simulink model "Full_Car_Model"  (R2023b)
settings: Solver=FixedStepAuto  StartTime=0.0  StopTime=t_end_sim  FixedStep=Ts_sim  RelTol=1e-3
values from neighbouring files (symbols this model uses):
  a_b_ref_sat = [ zeros(1,10) ... (first row only)    [A1_Init.m]    (also in C1_MonteCarloAnalysis.m)
  adaptive = 3    [A1_Init.m]    (also in C1_MonteCarloAnalysis.m = 1)
  data = A2_Full_car_model_parameters_4onBoard()    [A1_Init.m]    (also in C1_MonteCarloAnalysis.m)
  Ft_demand_F = [zeros(1,601) 200*ones(1,2400)]./data.R_F    [A1_Init.m]    (also in C1_MonteCarloAnalysis.m)
  Ft_demand_R = [zeros(1,(601-length(l_discr)))              200*ones(1,(2400+length(l_discr)))]./data.R_R    [A1_Init.m]    (also in C1_MonteCarloAnalysis.m)
  handmade_front = strcat(currentPath,'\Road_profiles\height_crg_files\','handmade_step_3cm_singlefunctions.crg')    [A1_Init.m]    (also in C1_MonteCarloAnalysis.m)
  handmade_mu_front = strcat(currentPath,'\Road_profiles\friction_crg_files\','handmade_fric_step_01_singlefunctions.crg')    [A1_Init.m]    (also in C1_MonteCarloAnalysis.m)
  handmade_mu_rear = handmade_mu_front    [A1_Init.m]    (also in C1_MonteCarloAnalysis.m)
  handmade_rear = handmade_front    [A1_Init.m]    (also in C1_MonteCarloAnalysis.m)
  LowLim_Q1 = -10    [A1_Init.m]    (also in C1_MonteCarloAnalysis.m)
  M = N    (= 10)    [A1_Init.m]    (also in C1_MonteCarloAnalysis.m)
  mu_distance = test_distance    [A1_Init.m]    (also in C1_MonteCarloAnalysis.m)
  mu_road = [ones(1,1001), 0.1*ones(1,2000)]    [A1_Init.m]    (also in C1_MonteCarloAnalysis.m)
  N = 10    [A1_Init.m]    (also in C1_MonteCarloAnalysis.m)
  N_iter = 3    [A1_Init.m]    (also in C1_MonteCarloAnalysis.m)
  omega_ini_F_L = x_u_dot_ini_F_L/data.R_F    [A1_Init.m]    (also in C1_MonteCarloAnalysis.m)
  omega_ini_F_R = x_u_dot_ini_R_R/data.R_F    [A1_Init.m]    (also in C1_MonteCarloAnalysis.m)
  omega_ini_R_L = x_u_dot_ini_R_L/data.R_R +2.483*1e-6    [A1_Init.m]    (also in C1_MonteCarloAnalysis.m)
  omega_ini_R_R = x_u_dot_ini_R_R/data.R_R+2.483*1e-6    [A1_Init.m]    (also in C1_MonteCarloAnalysis.m)
  passive = 2    [A1_Init.m]    (also in C1_MonteCarloAnalysis.m)
  Pitch = 0    [A1_Init.m]    (also in C1_MonteCarloAnalysis.m)
  Pitch_dot = 0    [A1_Init.m]    (also in C1_MonteCarloAnalysis.m)
  preview = 2    [A1_Init.m]    (also in C1_MonteCarloAnalysis.m)
  Q1 = 1e6    (= 1000000)    [A1_Init.m]    (also in C1_MonteCarloAnalysis.m)
  Q1_sat = 0    [A1_Init.m]    (also in C1_MonteCarloAnalysis.m)
  Q2 = 1e5    (= 100000)    [A1_Init.m]    (also in C1_MonteCarloAnalysis.m)
  QN1 = 0    [A1_Init.m]    (also in C1_MonteCarloAnalysis.m)
  QN2 = 0    [A1_Init.m]    (also in C1_MonteCarloAnalysis.m)
  R1 = 1e10    (= 10000000000)    [A1_Init.m]    (also in C1_MonteCarloAnalysis.m)
  r1_h0 = 0.99    [A1_Init.m]    (also in C1_MonteCarloAnalysis.m)
  r1_k = 1000    [A1_Init.m]    (also in C1_MonteCarloAnalysis.m)
  r1_max = 11    [A1_Init.m]    (also in C1_MonteCarloAnalysis.m)
  r1_min = -10    [A1_Init.m]    (also in C1_MonteCarloAnalysis.m)
  r2 = 2    [A1_Init.m]    (also in C1_MonteCarloAnalysis.m)
  R2 = 1e2    (= 100)    [A1_Init.m]    (also in C1_MonteCarloAnalysis.m)
  R2_rl = 2    [A1_Init.m]    (also in C1_MonteCarloAnalysis.m)
  road_profile = [zeros(1,801),ones(1,2200)*10*Step_selector]    [A1_Init.m]    (also in C1_MonteCarloAnalysis.m)
  T_distance = test_distance    [A1_Init.m]    (also in C1_MonteCarloAnalysis.m)
  T_hs_ini_F_L = 0    [A1_Init.m]    (also in C1_MonteCarloAnalysis.m)
  T_hs_ini_F_R = 0    [A1_Init.m]    (also in C1_MonteCarloAnalysis.m)
  T_hs_ini_R_L = 0    [A1_Init.m]    (also in C1_MonteCarloAnalysis.m)
  T_hs_ini_R_R = 0    [A1_Init.m]    (also in C1_MonteCarloAnalysis.m)
  test_distance = 0:0.01:30    [A1_Init.m]    (also in C1_MonteCarloAnalysis.m)
  theta_s_ini_F_L = 0    [A1_Init.m]    (also in C1_MonteCarloAnalysis.m)
  theta_s_ini_F_R = 0    [A1_Init.m]    (also in C1_MonteCarloAnalysis.m)
  theta_s_ini_R_L = 0    [A1_Init.m]    (also in C1_MonteCarloAnalysis.m)
  theta_s_ini_R_R = 0    [A1_Init.m]    (also in C1_MonteCarloAnalysis.m)
  theta_w_ini_F_L = -1.056*1e-2    (= -0.01056)    [A1_Init.m]    (also in C1_MonteCarloAnalysis.m)
  theta_w_ini_R_L = -1.056*1e-2    (= -0.01056)    [A1_Init.m]    (also in C1_MonteCarloAnalysis.m)
  Ts = 1e-3*[0 5 10 15 20 25 30 40 60 80 100]    [A1_Init.m]    (also in C1_MonteCarloAnalysis.m)
  w1_h0 = 0.0008    [A1_Init.m]    (also in C1_MonteCarloAnalysis.m)
  w1_k = 5000    [A1_Init.m]    (also in C1_MonteCarloAnalysis.m)
  w1_max = 9    [A1_Init.m]    (also in C1_MonteCarloAnalysis.m)
  w1_min = -10    [A1_Init.m]    (also in C1_MonteCarloAnalysis.m)
  w1_sat = 0.085    [A1_Init.m]    (also in C1_MonteCarloAnalysis.m)
  w2_h0 = 2    [A1_Init.m]    (also in C1_MonteCarloAnalysis.m)
  w2_inc = 0.05    [A1_Init.m]    (also in C1_MonteCarloAnalysis.m)
  w2_k = 10    [A1_Init.m]    (also in C1_MonteCarloAnalysis.m)
  w2_max = 5.3    [A1_Init.m]    (also in C1_MonteCarloAnalysis.m)
  w2_min = -10    [A1_Init.m]    (also in C1_MonteCarloAnalysis.m)
  Wmat_NMPC_init = [W(1,:) W(2,:) W(3,:) W(4,:)]    [A1_Init.m]    (also in C1_MonteCarloAnalysis.m)
  WNmat_NMPC_init = [WN(1,:) WN(2,:)]    [A1_Init.m]    (also in C1_MonteCarloAnalysis.m)
  X_0 = [z_b_dot_ini z_b_ini z_u_dot_ini_F_L z_u_ini_F_L x_b_dot_ini x_b_ini x_u_dot_ini_F_L x_u_ini_F_L          omega_ini_F_L theta_w_ini_F_L omega_ini_F_L theta_s_ini_F_L torque_ini_F_L]    [A1_Init.m]    (also in C1_MonteCarloAnalysis.m)
  x_b_dot_ini = speed_ini/3.6    (= 11.1111111111)    [A1_Init.m]    (also in C1_MonteCarloAnalysis.m)
  x_b_ini = data.b+pos_ini    [A1_Init.m]    (also in C1_MonteCarloAnalysis.m)
  x_u_dot_ini_F_L = speed_ini/3.6 - 1.125*1e-4    (= 11.1109986111)    [A1_Init.m]    (also in C1_MonteCarloAnalysis.m)
  x_u_dot_ini_F_R = speed_ini/3.6 - 1.125*1e-4    (= 11.1109986111)    [A1_Init.m]    (also in C1_MonteCarloAnalysis.m)
  x_u_dot_ini_R_L = speed_ini/3.6 - 1.125*1e-4    (= 11.1109986111)    [A1_Init.m]    (also in C1_MonteCarloAnalysis.m)
  x_u_dot_ini_R_R = speed_ini/3.6 - 1.125*1e-4    (= 11.1109986111)    [A1_Init.m]    (also in C1_MonteCarloAnalysis.m)
  x_u_ini_F_L = data.a+data.b+pos_ini    [A1_Init.m]    (also in C1_MonteCarloAnalysis.m)
  x_u_ini_F_R = data.a+data.b+pos_ini    [A1_Init.m]    (also in C1_MonteCarloAnalysis.m)
  x_u_ini_R_L = pos_ini    (= 0)    [A1_Init.m]    (also in C1_MonteCarloAnalysis.m)
  x_u_ini_R_R = pos_ini    (= 0)    [A1_Init.m]    (also in C1_MonteCarloAnalysis.m)
  z_b_dot_ini = 0    [A1_Init.m]    (also in C1_MonteCarloAnalysis.m)
  z_b_ini = 0    [A1_Init.m]    (also in C1_MonteCarloAnalysis.m)
  z_u_dot_ini_F_L = 0    [A1_Init.m]    (also in C1_MonteCarloAnalysis.m)
  z_u_dot_ini_F_R = 0    [A1_Init.m]    (also in C1_MonteCarloAnalysis.m)
  z_u_dot_ini_R_L = 0    [A1_Init.m]    (also in C1_MonteCarloAnalysis.m)
  z_u_dot_ini_R_R = 0    [A1_Init.m]    (also in C1_MonteCarloAnalysis.m)
  z_u_ini_F_L = 0    [A1_Init.m]    (also in C1_MonteCarloAnalysis.m)
  z_u_ini_F_R = 0    [A1_Init.m]    (also in C1_MonteCarloAnalysis.m)
  z_u_ini_R_L = 0    [A1_Init.m]    (also in C1_MonteCarloAnalysis.m)
  z_u_ini_R_R = 0    [A1_Init.m]    (also in C1_MonteCarloAnalysis.m)
undefined symbols (not defined in the file or in its folder): Delay_step, road_with_noise
libraries: mfswift_library x8, rllib x4, simulink x4
(part 6 of 7)

== matlab function Full_Car_Model/CONTROLLER REAR RIGHT/ROAD PREVIEW/ROAD PREVIEW ==
  data: w input; OnlineData output; beta_y input; Tm_req input; Tm_req_R2 input; Tm_req_F_L input; Tm_req_F_R input; N parameter; M parameter; mu_act input; sigma_ref input
function OnlineData=OnlineDataArray(w, beta_y, Tm_req, Tm_req_R2, Tm_req_F_L, Tm_req_F_R, N, M, mu_act, sigma_ref)

OnlineData = repmat([0; 0; Tm_req; Tm_req_R2; Tm_req_F_L; Tm_req_F_R; 0; 0],N+1,1);

for i = 1:M+1       % M = Time preview steps
    OnlineData(8*i-7) = w(i);
    OnlineData(8*i-6) = beta_y(i);
    OnlineData(8*i-1) = mu_act(i);
    OnlineData(8*i) = sigma_ref(i);
end

for i = M+2:N+1     % N = Time horizon steps
    OnlineData(8*i-7) = w(end);
    OnlineData(8*i-6) = beta_y(end);
    OnlineData(8*i-1) = mu_act(end);
    OnlineData(8*i) = sigma_ref(end);
%}
end

== matlab function Full_Car_Model/PLANT MODEL WITH MF-SWIFT/SUSPENSION MODEL/Anti-properties ==
  data: x_b_ddot input; Fz_unsprung_F output; data parameter; Fz_unsprung_R output; delta_F_z_AP output; delta_M_z_AP output
function [Fz_unsprung_F, Fz_unsprung_R, delta_F_z_AP, delta_M_z_AP] = fcn(x_b_ddot, data)

% Hypothesis: front to total = 50 % ----> calculate it in a future
% implementation
AP_F    = data.AP_F;   % Anti properties percentage
AP_R    = data.AP_R;   % Anti properties percentage
p_inst  = data.p_inst; % Anti properties percentage

p = 0.5;

fi_F  = atan(AP_F*data.hg/(p_inst*data.L));       % in order to have anti = 5 %
fi_R  = atan(AP_R*data.hg/((1 - p_inst)*data.L)); % in order to have anti = 5 %

delta_F_zF  = +(data.m_b + data.m_u_F + data.m_u_R)*x_b_ddot*data.hg/data.L...
              -(data.m_b + data.m_u_F + data.m_u_R)*x_b_ddot*tan(fi_F)*p;
delta_F_zR  = -(data.m_b + data.m_u_F + data.m_u_R)*x_b_ddot*data.hg/data.L...
              +(data.m_b + data.m_u_F + data.m_u_R)*x_b_ddot*tan(fi_R)*(1-p);

Fz_unsprung_F  = -(data.m_b + data.m_u_F + data.m_u_R)*x_b_ddot*tan(fi_F)*p;
Fz_unsprung_R  = +(data.m_b + data.m_u_F + data.m_u_R)*x_b_ddot*tan(fi_R)*(1-p);

delta_F_z_AP  = delta_F_zF + delta_F_zR;
delta_M_z_AP  = delta_F_zF*data.a - delta_F_zR*data.b;

== matlab function Full_Car_Model/CONTROLLER REAR LEFT/MATLAB Function ==
  data: z_b_dot input; z_b_dot_R output; z_b input; z_u_dot_R_L input; z_u_R_L input; x_b_dot input; x_b input; x_u_dot_R_L input; x_u_R_L input; theta_w_dot input; theta_w input; theta_s_dot input; theta_s input; z_b_R output; z_u_dot_R_L output; z_u_R_L output; x_b_dot_R output; x_b_R output; x_u_dot_R_L output; x_u_R_L output; theta_w_dot output; theta_w output; theta_s_dot output; theta_s output; torque input; torque output; pitch_dot input; pitch input; b input
function [z_b_dot_R, z_b_R, z_u_dot_R_L, z_u_R_L,...
          x_b_dot_R, x_b_R, x_u_dot_R_L, x_u_R_L,...
          theta_w_dot, theta_w, theta_s_dot, theta_s, torque]...
          = fcn(z_b_dot, z_b, z_u_dot_R_L, z_u_R_L,...
                x_b_dot, x_b, x_u_dot_R_L, x_u_R_L,...
                theta_w_dot, theta_w, theta_s_dot, theta_s, torque,...
                pitch_dot, pitch, b)

z_b_dot_R   = z_b_dot - pitch_dot*b;
z_b_R       = z_b - b*pitch;
x_b_dot_R   = x_b_dot;
x_b_R       = x_b - b;

end

== matlab function Full_Car_Model/CONTROLLER REAR LEFT/ROAD PREVIEW/NO_ROAD_PREVIEW ==
  data: w input; OnlineData output; Tm_req input; Tm_req_R2 input; Tm_req_F_L input; Tm_req_F_R input; N parameter; mu_act input; sigma_ref input
function OnlineData=OnlineDataArray(w, Tm_req, Tm_req_R2, Tm_req_F_L, Tm_req_F_R, N, mu_act, sigma_ref)

OnlineData = repmat([w; 0; Tm_req; Tm_req_R2; Tm_req_F_L; Tm_req_F_R; mu_act; sigma_ref],N+1,1);
end

== matlab function Full_Car_Model/CONTROLLER REAR RIGHT/ROAD PREVIEW/Time-based Road Preview/MATLAB Function2 ==
  data: z_road input; Z_ef output; Z_er output; data parameter; M parameter
function [Z_ef, Z_er] = fcn(z_road, data, M)

n_ellipse_width = length(-data.ac:0.01:data.ac);
x_ef = -data.ac:data.ac_step:data.ac;
x_er = x_ef;

Z_ef = zeros(M+1,1);
Z_er = zeros(M+1,1);
for i = 1:M+1
    Z_ef(i) = max(z_road(i,end-n_ellipse_width+1:end) + abs(data.bc*(1-(abs(x_ef)/data.ac).^data.c).^(1/data.c)));
    Z_er(i) = max(z_road(i,1:n_ellipse_width) + abs(data.bc*(1-(abs(x_er)/data.ac).^data.c).^(1/data.c)));
end

== matlab function Full_Car_Model/CONTROLLER REAR RIGHT/ROAD PREVIEW/Time-based Road Preview/MATLAB Function3 ==
  data: Z_ef input; w output; Z_er input; beta_y output; data parameter; M parameter
function [w, beta_y] = fcn(Z_ef, Z_er,data, M)

w      = zeros(M+1,1);
beta_y = zeros(M+1,1);

for i = 1:M+1
    w(i) = (Z_ef(i) + Z_er(i))/2 - data.bc;
    beta_y(i) = atan((Z_ef(i) - Z_er(i))/data.ls);
end

== matlab function Full_Car_Model/CONTROLLER REAR LEFT/ROAD PREVIEW/ROAD PREVIEW ==
  data: w input; OnlineData output; beta_y input; Tm_req input; Tm_req_R2 input; Tm_req_F_L input; Tm_req_F_R input; N parameter; M parameter; mu_act input; sigma_ref input
function OnlineData=OnlineDataArray(w, beta_y, Tm_req, Tm_req_R2, Tm_req_F_L, Tm_req_F_R, N, M, mu_act, sigma_ref)

OnlineData = repmat([0; 0; Tm_req; Tm_req_R2; Tm_req_F_L; Tm_req_F_R; 0; 0],N+1,1);

for i = 1:M+1       % M = Time preview steps
    OnlineData(8*i-7) = w(i);
    OnlineData(8*i-6) = beta_y(i);
    OnlineData(8*i-1) = mu_act(i);
    OnlineData(8*i) = sigma_ref(i);
end

for i = M+2:N+1     % N = Time horizon steps
    OnlineData(8*i-7) = w(end);
    OnlineData(8*i-6) = beta_y(end);
    OnlineData(8*i-1) = mu_act(end);
    OnlineData(8*i) = sigma_ref(end);
%}
end

== matlab function Full_Car_Model/CONTROLLER REAR RIGHT/ROAD PREVIEW/Time-based Road Preview/MATLAB Function6 ==
  data: X_i input; X_road output; M parameter; data parameter
function X_road = fcn(X_i, M, data)

n = length(0:0.01:data.ac*2+data.ls);

X_road = zeros(M+1, n+1);

for i=1:M+1
    for j=1:1:n+1
        X_road(i,j) = X_i(i) - data.ls/2 - data.ac + data.ac_step*(j-1);
    end
end

== matlab function Full_Car_Model/CONTROLLER REAR RIGHT/ROAD PREVIEW/Time-based Road Preview/X(i)1 ==
  data: X_i output; X_u_current input; x_u_dot_current input; Ts parameter; M parameter
function X_i= fcn(X_u_current, x_u_dot_current, Ts, M)

X_i = zeros(M+1,1);

for i=1:M+1
    X_i(i) = X_u_current + x_u_dot_current * Ts(i);
end

== matlab function Full_Car_Model/CONTROLLER FRONT LEFT/ROAD PREVIEW/ROAD PREVIEW ==
  data: w input; OnlineData output; beta_y input; Tm_req input; Tm_req_F2 input; Tm_req_R_L input; Tm_req_R_R input; N parameter; M parameter; mu_act input; sigma_ref input
function OnlineData=OnlineDataArray(w, beta_y, Tm_req, Tm_req_F2, Tm_req_R_L, Tm_req_R_R, N, M, mu_act, sigma_ref)

OnlineData = repmat([0; 0; Tm_req; Tm_req_F2; Tm_req_R_L; Tm_req_R_R; 0; 0],N+1,1);

for i = 1:M+1       % M = Time preview steps
    OnlineData(8*i-7) = w(i);
    OnlineData(8*i-6) = beta_y(i);
    OnlineData(8*i-1) = mu_act(i);
    OnlineData(8*i) = sigma_ref(i);
end

for i = M+2:N+1     % N = Time horizon steps
    OnlineData(8*i-7) = w(end);
    OnlineData(8*i-6) = beta_y(end);
    OnlineData(8*i-1) = mu_act(end);
    OnlineData(8*i) = sigma_ref(end);

end

== matlab function Full_Car_Model/NMPC Internal model FL/MATLAB Function1 ==
  data: z_b_ddot output; z_u_ddot output; x_b_ddot output; x_u_ddot output; States input size=13; road input; Tm_req_F2 input; Tm_req_R_L input; Tm_req_R_R input; theta_w_ddot output; theta_s_ddot output; mu_act input; data parameter

function [z_b_ddot, z_u_ddot, x_b_ddot, x_u_ddot, theta_w_ddot, theta_s_ddot] =...
    InternalModelNMPC(States, road, Tm_req_F2, Tm_req_R_L, Tm_req_R_R, mu_act, data)

x_b_dot     = States(1);
x_b         = States(2);
x_u_dot     = States(3);
x_u         = States(4);
z_b_dot     = States(5);
z_b         = States(6);
z_u_dot     = States(7);
z_u         = States(8);
theta_w_dot = States(9);
theta_w     = States(10);
theta_s_dot = States(11);
theta_s     = States(12);
torque      = States(13);

w           = road(1);
beta_y      = road(2);

%% relative displacement and speed
epsilon_dot_x   = (x_b_dot - x_u_dot);        % Longitudinal relative speed
epsilon_dot_z   = (z_b_dot - z_u_dot);        % Vertical relative speed

epsilon_x       = (x_b - x_u);                % Longitudinal relative displacement
epsilon_z       = (z_b - z_u);                % Vertical relative displacement

%% Vertical damper force
Fc_x = (data.c_x_F * epsilon_dot_x);
Fc_z = (0.71*(400*(-1.5 + atan(10*0.71*epsilon_dot_z + 0.1)/(pi/2))...
     + 1400*(1 + atan(18*0.71*epsilon_dot_z - 1.4)/(pi/2))));

Fk_x = (data.k_x_F * epsilon_x);
Fk_z = (data.k_z_F * epsilon_z);

%% Inverse tyre model equations
Fr_x = ((w - z_u)*cos(beta_y) * data.k_r_F * sin(beta_y));
Fr_z = ((w - z_u)*cos(beta_y) * data.k_r_F * cos(beta_y));

Ft_x = ((w - z_u)*sin(beta_y) * data.k_t_F * 5 * cos(beta_y));
Ft_z = ((w - z_u)*sin(beta_y) * data.k_t_F * 5 * sin(beta_y));

%% Longitudinal dynamics - Drag forces
F_drag = (data.Aero_Coeff * x_b_dot^2);

%% Rolling resistance - Front
f_roll_F = (data.f_0_F + data.f_2_F*x_b_dot^2);
F_roll_F = (f_roll_F * data.m_total * data.b/data.L * data.g);

%% Rolling resistance - Rear
f_roll_R = (data.f_0_R + data.f_2_R*x_b_dot^2);
F_roll_R = (f_roll_R * data.m_total * data.a/data.L * data.g);

%% Deflection of the tyre
delta_rho = ((w - z_u)*cos(beta_y));
rho = (0.3833 - 0.5*data.m_total*9.81*data.b/data.L/data.k_r_F - delta_rho); % - m_total*9.81*b/L/k_r

%% Pacejka
sigma_th        = (1-(x_u_dot/(theta_w_dot*data.R_F)));       % Longitudinal slip
F_z             = ((Fr_z + 0.5*data.m_total*9.81*data.b/data.L));     % N     

% --------------------------------------------------------------------------
% Longitudinal Equation at pure slip - FxTyreFL
% --------------------------------------------------------------------------
gamma_x = data.gammaFL * data.LGAX;
dfz     = ((F_z - data.LFZO*data.FZ0)/(data.LFZO*data.FZ0));
mu      = ((mu_act+1e-10) * (data.PDX1 + data.PDX2* dfz)*( 1 - data.PDX3 * gamma_x^2 ).*data.LMUX);
SHx     = ((data.PHX1 + data.PHX2 * dfz)*data.LHX);
sigma_x = (sigma_th + SHx);
C       = data.PCX1 * data.LCX;
D       = (mu * F_z);
E       = ((data.PEX1 + data.PEX2*dfz + data.PEX3 * dfz^2).*data.LEX);

Kx      = (F_z * (data.PKX1 + data.PKX2 * dfz) * 2.71828^(data.PKX3 * dfz) * data.LKX);
Svx     = (F_z * ( data.PVX1 + data.PVX2 * dfz ) * data.LVX * data.LMUX * data.mu_max);
B       = (Kx/(C*D));
F_x     = (D * sin(C*atan(B*sigma_x - E*(B*sigma_x - atan( B* sigma_x )))) + Svx);
Fx_x    = (F_x*cos(beta_y));
Fx_z    = (F_x*sin(beta_y));

%% HALF SHAFT EQUATIONS

fa = (data.k_hs_F4*(theta_s - theta_w + data.backlash_F4)); %
fb = (data.k_hs_F4*(theta_s - theta_w - data.backlash_F4)); %
fc = (data.b_hs_F4*(theta_s_dot - theta_w_dot));
f2_exp = (exp(2*data.a_diff*( data.backlash_F4 - (theta_s - theta_w)))); %
f1_exp = (exp(2*data.a_diff*( data.backlash_F4 + (theta_s - theta_w)))); %
f1 = (0.5*((1-f1_exp) / (1+f1_exp)) + 0.5);
f2 = (0.5*((1-f2_exp) / (1+f2_exp)) + 0.5);

T_hs_K = (fa*f1 + fb*f2);
T_hs_B = (fc*f1 + fc*f2);

T_hs = (T_hs_K + T_hs_B);

T_t = (data.i_t_F4*data.n_t_F4*torque);

%% Quarter-car model equations
z_b_ddot    = ((- Fk_z - Fc_z)/(data.m_b*data.b/(data.L*2))); 

z_u_ddot    = ((  Fk_z + Fc_z + Fr_z - Ft_z + Fx_z)/data.m_u_F);        

x_b_ddot    = ((- Fk_x - Fc_x...
            + Tm_req_F2/data.R_F + Tm_req_R_R/data.R_R +Tm_req_R_L/data.R_R...
            - F_drag - 0.5*F_roll_F - F_roll_R)/data.m_app_FL);

x_u_ddot    = ((Fk_x + Fc_x - Fr_x - Ft_x + Fx_x)/data.m_u_F);

MyFL0       = (rho * (F_z).* (data.QSY1 + data.QSY2 * (F_z)./data.FNOMIN));

theta_w_ddot   = ((T_hs - F_x*rho - MyFL0)/data.I_y_F);

theta_s_ddot = (T_t - T_hs) / data.J_eq_F4;

== matlab function Full_Car_Model/CONTROLLER FRONT LEFT/ROAD PREVIEW/Time-based Road Preview/MATLAB Function1 ==
  data: z_road input; Z_ef output; Z_er output; data parameter; M parameter
function [Z_ef, Z_er] = fcn(z_road, data, M)

n_ellipse_width = length(-data.ac:0.01:data.ac);
x_ef = -data.ac:data.ac_step:data.ac;
x_er = x_ef;

Z_ef = zeros(M+1,1);
Z_er = zeros(M+1,1);
for i = 1:M+1
    Z_ef(i) = max(z_road(i,end-n_ellipse_width+1:end) + abs(data.bc*(1-(abs(x_ef)/data.ac).^data.c).^(1/data.c)));
    Z_er(i) = max(z_road(i,1:n_ellipse_width) + abs(data.bc*(1-(abs(x_er)/data.ac).^data.c).^(1/data.c)));
end

== matlab function Full_Car_Model/CONTROLLER FRONT LEFT/ROAD PREVIEW/Time-based Road Preview/MATLAB Function4 ==
  data: Z_ef input; w output; Z_er input; beta_y output; data parameter; M parameter
function [w, beta_y] = fcn(Z_ef, Z_er,data, M)

w      = zeros(M+1,1);
beta_y = zeros(M+1,1);

for i = 1:M+1
    w(i) = (Z_ef(i) + Z_er(i))/2 - data.bc;
    beta_y(i) = atan((Z_ef(i) - Z_er(i))/data.ls);
end

== matlab function Full_Car_Model/CONTROLLER FRONT LEFT/ROAD PREVIEW/Time-based Road Preview/MATLAB Function5 ==
  data: X_i input; X_road output; M parameter; data parameter
function X_road = fcn(X_i, M, data)

n = length(0:0.01:data.ac*2+data.ls);

X_road = zeros(M+1, n+1);

for i=1:M+1
    for j=1:1:n+1
        X_road(i,j) = X_i(i) - data.ls/2 - data.ac + data.ac_step*(j-1);
    end
end

== matlab function Full_Car_Model/CONTROLLER FRONT LEFT/ROAD PREVIEW/Time-based Road Preview/X(i)1 ==
  data: X_i output; X_u_current input; x_u_dot_current input; Ts parameter; M parameter
function X_i= fcn(X_u_current, x_u_dot_current, Ts, M)

X_i = zeros(M+1,1);

for i=1:M+1
    X_i(i) = X_u_current + x_u_dot_current * Ts(i);
end

== matlab function Full_Car_Model/CONTROLLER FRONT LEFT/Rule based/MATLAB Function2 ==
  data: dT_req input; W output; w2_min parameter; w2_max parameter; w2_k parameter; w2_h0 parameter; mu input; w2_inc parameter
function W = fcn(dT_req, w2_min, w2_max, w2_k, w2_h0, mu, w2_inc)
h=0;

x1 = linspace(0, 1, length(dT_req));
exp_decay = exp(5 * x1) - 1;  
perc = exp_decay / sum(exp_decay);

for i=1:length(dT_req)
    h=h+dT_req(i)*perc(i);
end
W=w2_min+(w2_max-w2_min)/(1+exp(-w2_k*(abs(h)-w2_h0)));

% The larger is w2_inc, the more W is incremented
W = (W - w2_min)/(mu^w2_inc) + w2_min;

== matlab function Full_Car_Model/CONTROLLER FRONT LEFT/Rule based/MATLAB Function3 ==
  data: flag input; mu_prev input; W output; M parameter; r1_min parameter; r1_max parameter; r1_k parameter; r1_h0 parameter
function W = fcn(flag, mu_prev,M, r1_min, r1_max, r1_k, r1_h0)
h=0; 

x2 = linspace(0, 1, M+1);    
exp_growth = exp(1 * x2) - 1;  

perc = exp_growth; 
perc = perc / sum(perc);

for i=1:M+1
    h=h+mu_prev(i)*perc(i);
end

W=r1_min+(r1_max-r1_min)/(1+exp(r1_k*(abs(h)-r1_h0)));

if not(flag)
    W = r1_min;
end

== matlab function Full_Car_Model/CONTROLLER FRONT LEFT/Weight matrixes/MATLAB Function ==
  data: Q1 input; Wmat_NMPC output; Q2 input; QN1 input; QN2 input; R1 input; R2 input; WNmat_NMPC output
function [Wmat_NMPC,WNmat_NMPC] = fcn(Q1, Q2, QN1, QN2, R1, R2) 
W                   = diag([Q1 Q2 R1 R2]);
WN                  = diag([QN1 QN2]);
Wmat_NMPC   = [W(1,:) W(2,:) W(3,:) W(4,:)]';
WNmat_NMPC  = [WN(1,:) WN(2,:)]';
end

== matlab function Full_Car_Model/CONTROLLER FRONT LEFT/Rule based/Subsystem/MATLAB Function ==
  data: OnlineData input; w output; M parameter; mu_act output
function [w, mu_act]=fcn(OnlineData, M)

w=zeros(M+1,1);
mu_act=zeros(M+1,1);

for i = 1:M+1       % M = Time preview steps
    w(i) = OnlineData(8*i-7);
    mu_act(i) = OnlineData(8*i-1);
end

== matlab function Full_Car_Model/CONTROLLER FRONT LEFT/MATLAB Function1 ==
  data: Wmat_NMPC input; cost_fcn_weights output
function cost_fcn_weights = fcn(Wmat_NMPC) 
    cost_fcn_weights = Wmat_NMPC(1:5:end);
end

== matlab function Full_Car_Model/CONTROLLER REAR LEFT/MATLAB Function1 ==
  data: Wmat_NMPC input; cost_fcn_weights output
function cost_fcn_weights = fcn(Wmat_NMPC) 
    cost_fcn_weights = Wmat_NMPC(1:5:end);
end

== matlab function Full_Car_Model/CONTROLLER REAR LEFT/Rule based/MATLAB Function ==
  data: w_prev input; W output; w1_h0 parameter; w1_k parameter; w1_max parameter; w1_min parameter; mu input; w1_sat parameter
function W = fcn(w_prev,w1_h0, w1_k, w1_max, w1_min, mu, w1_sat)
h=0;

w_var=zeros(1,length(w_prev)-1);

x1 = linspace(0, 1, length(w_prev)-1);
exp_growth = exp(1 * x1) - 1;   
perc = exp_growth / sum(exp_growth);

for i=1:length(w_prev)-1
    w_var(i)=abs(w_prev(i+1)-w_prev(i)); 
    h=h+w_var(i)*perc(i);
end
W=w1_min+(w1_max-w1_min)/(1+exp(-w1_k*(abs(h)-w1_h0)));

% Saturation between - w1_min and W. The larger is w1_sat, the more is saturated
W = (W - w1_min)*mu^w1_sat + w1_min;

== matlab function Full_Car_Model/CONTROLLER REAR LEFT/Rule based/MATLAB Function2 ==
  data: dT_req input; W output; w2_min parameter; w2_max parameter; w2_k parameter; w2_h0 parameter; mu input; w2_inc parameter
function W = fcn(dT_req, w2_min, w2_max, w2_k, w2_h0, mu, w2_inc)
h=0;

x1 = linspace(0, 1, length(dT_req));
exp_decay = exp(5 * x1) - 1;  
perc = exp_decay / sum(exp_decay);

for i=1:length(dT_req)
    h=h+dT_req(i)*perc(i);
end
W=w2_min+(w2_max-w2_min)/(1+exp(-w2_k*(abs(h)-w2_h0)));

% The larger is w2_inc, the more W is incremented
W = (W - w2_min)/(mu^w2_inc) + w2_min;

== matlab function Full_Car_Model/CONTROLLER FRONT LEFT/RL_weights/Subsystem2/MATLAB Function ==
  data: OnlineData input; w output; M parameter; mu_act output; sigma_ref output
function [w, mu_act, sigma_ref]=fcn(OnlineData, M)

w=zeros(M+1,1);
mu_act=zeros(M+1,1);
sigma_ref=zeros(M+1,1);

for i = 1:M+1       % M = Time preview steps
    w(i) = OnlineData(8*i-7);
    mu_act(i) = OnlineData(8*i-1);
    sigma_ref(i) = OnlineData(8*i);
end

== matlab function Full_Car_Model/CONTROLLER REAR LEFT/ROAD PREVIEW/Time-based Road Preview/MATLAB Function2 ==
  data: z_road input; Z_ef output; Z_er output; data parameter; M parameter
function [Z_ef, Z_er] = fcn(z_road, data, M)

n_ellipse_width = length(-data.ac:0.01:data.ac);
x_ef = -data.ac:data.ac_step:data.ac;
x_er = x_ef;

Z_ef = zeros(M+1,1);
Z_er = zeros(M+1,1);
for i = 1:M+1
    Z_ef(i) = max(z_road(i,end-n_ellipse_width+1:end) + abs(data.bc*(1-(abs(x_ef)/data.ac).^data.c).^(1/data.c)));
    Z_er(i) = max(z_road(i,1:n_ellipse_width) + abs(data.bc*(1-(abs(x_er)/data.ac).^data.c).^(1/data.c)));
end

== matlab function Full_Car_Model/CONTROLLER REAR LEFT/ROAD PREVIEW/Time-based Road Preview/MATLAB Function3 ==
  data: Z_ef input; w output; Z_er input; beta_y output; data parameter; M parameter
function [w, beta_y] = fcn(Z_ef, Z_er,data, M)

w      = zeros(M+1,1);
beta_y = zeros(M+1,1);

for i = 1:M+1
    w(i) = (Z_ef(i) + Z_er(i))/2 - data.bc;
    beta_y(i) = atan((Z_ef(i) - Z_er(i))/data.ls);
end

== matlab function Full_Car_Model/CONTROLLER REAR LEFT/ROAD PREVIEW/Time-based Road Preview/MATLAB Function6 ==
  data: X_i input; X_road output; M parameter; data parameter
function X_road = fcn(X_i, M, data)

n = length(0:0.01:data.ac*2+data.ls);

X_road = zeros(M+1, n+1);

for i=1:M+1
    for j=1:1:n+1
        X_road(i,j) = X_i(i) - data.ls/2 - data.ac + data.ac_step*(j-1);
    end
end

== matlab function Full_Car_Model/NMPC Internal model FL/Time-based Road Preview/MATLAB Function5 ==
  data: X input; x_road output; M parameter; data parameter
function x_road = fcn(X, M, data)

n = length(0:0.01:data.ac*2+data.ls);

% cams_projection = 85;  % ls+2*ac

d_step = 0.01; %1 cm

x_road = zeros(n+1,1);

for i=1:1:n+1
    x_road(i) = X - data.ls/2 - data.ac + d_step*(i-1);
end

== matlab function Full_Car_Model/CONTROLLER REAR LEFT/ROAD PREVIEW/Time-based Road Preview/X(i)1 ==
  data: X_i output; X_u_current input; x_u_dot_current input; Ts parameter; M parameter
function X_i= fcn(X_u_current, x_u_dot_current, Ts, M)

X_i = zeros(M+1,1);

for i=1:M+1
    X_i(i) = X_u_current + x_u_dot_current * Ts(i);
end

== matlab function Full_Car_Model/CONTROLLER FRONT RIGHT/RL_weights/Subsystem2/MATLAB Function ==
  data: OnlineData input; w output; M parameter; mu_act output; sigma_ref output
function [w, mu_act, sigma_ref]=fcn(OnlineData, M)

w=zeros(M+1,1);
mu_act=zeros(M+1,1);
sigma_ref=zeros(M+1,1);

for i = 1:M+1       % M = Time preview steps
    w(i) = OnlineData(8*i-7);
    mu_act(i) = OnlineData(8*i-1);
    sigma_ref(i) = OnlineData(8*i);
end

== matlab function Full_Car_Model/CONTROLLER REAR LEFT/RL_weights/MATLAB Function ==
  data: w_prev input; h output; M parameter
function h = fcn(w_prev,M)
h=0;   
w1_memo=5;
w_var=zeros(1,M+w1_memo+1);

x1 = linspace(0, 1, w1_memo);         
x2 = linspace(1, 0, M+1); 
exp_growth = exp(1 * x1) - 1;   
exp_decay = exp(1 * x2) - 1;  

perc = [exp_growth, exp_decay]; 
perc = perc / sum(perc);

for i=1:M+w1_memo
    w_var(i)=w_prev(i+1)-w_prev(i); 
    h=h+w_var(i)*perc(i);
end

== matlab function Full_Car_Model/CONTROLLER REAR LEFT/RL_weights/MATLAB Function3 ==
  data: mu_prev input; h output; M parameter
function h = fcn(mu_prev,M)
h=0; 

x2 = linspace(1, 0, M+1);    
exp_decay = exp(1 * x2) - 1;  

perc = exp_decay; 
perc = perc / sum(perc);

for i=1:M+1
    h=h+mu_prev(i)*perc(i);
end

== matlab function Full_Car_Model/CONTROLLER REAR RIGHT/RL_weights/MATLAB Function ==
  data: w_prev input; h output; M parameter
function h = fcn(w_prev,M)
h=0;   
w1_memo=5;
w_var=zeros(1,M+w1_memo+1);

x1 = linspace(0, 1, w1_memo);         
x2 = linspace(1, 0, M+1); 
exp_growth = exp(1 * x1) - 1;   
exp_decay = exp(1 * x2) - 1;  

perc = [exp_growth, exp_decay]; 
perc = perc / sum(perc);

for i=1:M+w1_memo
    w_var(i)=w_prev(i+1)-w_prev(i); 
    h=h+w_var(i)*perc(i);
end

== matlab function Full_Car_Model/CONTROLLER REAR LEFT/RL_weights/Subsystem2/MATLAB Function ==
  data: OnlineData input; w output; M parameter; mu_act output; sigma_ref output
function [w, mu_act, sigma_ref]=fcn(OnlineData, M)

w=zeros(M+1,1);
mu_act=zeros(M+1,1);
sigma_ref=zeros(M+1,1);

for i = 1:M+1       % M = Time preview steps
    w(i) = OnlineData(8*i-7);
    mu_act(i) = OnlineData(8*i-1);
    sigma_ref(i) = OnlineData(8*i);
end

== matlab function Full_Car_Model/CONTROLLER FRONT LEFT/RL_weights/MATLAB Function3 ==
  data: mu_prev input; h output; M parameter
function h = fcn(mu_prev,M)
h=0; 

x2 = linspace(1, 0, M+1);    
exp_decay = exp(1 * x2) - 1;  

perc = exp_decay; 
perc = perc / sum(perc);

for i=1:M+1
    h=h+mu_prev(i)*perc(i);
end

== matlab function Full_Car_Model/CONTROLLER REAR RIGHT/RL_weights/MATLAB Function3 ==
  data: mu_prev input; h output; M parameter
function h = fcn(mu_prev,M)
h=0; 

x2 = linspace(1, 0, M+1);    
exp_decay = exp(1 * x2) - 1;  

perc = exp_decay; 
perc = perc / sum(perc);

for i=1:M+1
    h=h+mu_prev(i)*perc(i);
end

== matlab function Full_Car_Model/CONTROLLER REAR RIGHT/RL_weights/Subsystem2/MATLAB Function ==
  data: OnlineData input; w output; M parameter; mu_act output; sigma_ref output
function [w, mu_act, sigma_ref]=fcn(OnlineData, M)

w=zeros(M+1,1);
mu_act=zeros(M+1,1);
sigma_ref=zeros(M+1,1);

for i = 1:M+1       % M = Time preview steps
    w(i) = OnlineData(8*i-7);
    mu_act(i) = OnlineData(8*i-1);
    sigma_ref(i) = OnlineData(8*i);
end

== matlab function Full_Car_Model/CONTROLLER FRONT RIGHT/Subsystem1/MATLAB Function ==
  data: Q1 input; Wmat_NMPC output; Q2 input; R1 input; R2 input
function Wmat_NMPC = fcn(Q1, Q2, R1, R2) 
     W = diag([Q1 Q2 R1 R2]);
     Wmat_NMPC   = [W(1,:) W(2,:) W(3,:) W(4,:)]';
    % W = diag([Q1 R1 R2]);
    % Wmat_NMPC   = [W(1,:) W(2,:) W(3,:)]';
end

== matlab function Full_Car_Model/CONTROLLER FRONT RIGHT/Subsystem1/MATLAB Function1 ==
  data: QN1 input; WNmat_NMPC output; QN2 input
function WNmat_NMPC = fcn(QN1, QN2) 
     WN                  = diag([QN1 QN2]);
     WNmat_NMPC  = [WN(1,:) WN(2,:)]'; 
    % WN                  = diag([QN1]);
    % WNmat_NMPC  = [WN(1,:) WN(2,:)]'; 
end

== matlab function Full_Car_Model/CONTROLLER REAR LEFT/Subsystem1/MATLAB Function ==
  data: Q1 input; Wmat_NMPC output; Q2 input; R1 input; R2 input
function Wmat_NMPC = fcn(Q1, Q2, R1, R2) 
     W = diag([Q1 Q2 R1 R2]);
     Wmat_NMPC   = [W(1,:) W(2,:) W(3,:) W(4,:)]';
    % W = diag([Q1 R1 R2]);
    % Wmat_NMPC   = [W(1,:) W(2,:) W(3,:)]';
end

== matlab function Full_Car_Model/CONTROLLER REAR LEFT/Subsystem1/MATLAB Function1 ==
  data: QN1 input; WNmat_NMPC output; QN2 input
function WNmat_NMPC = fcn(QN1, QN2) 
     WN                  = diag([QN1 QN2]);
     WNmat_NMPC  = [WN(1,:) WN(2,:)]'; 
    % WN                  = diag([QN1]);
    % WNmat_NMPC  = [WN(1,:) WN(2,:)]'; 
end

== matlab function Full_Car_Model/CONTROLLER REAR RIGHT/Subsystem1/MATLAB Function ==
  data: Q1 input; Wmat_NMPC output; Q2 input; R1 input; R2 input
function Wmat_NMPC = fcn(Q1, Q2, R1, R2) 
     W = diag([Q1 Q2 R1 R2]);
     Wmat_NMPC   = [W(1,:) W(2,:) W(3,:) W(4,:)]';
    % W = diag([Q1 R1 R2]);
    % Wmat_NMPC   = [W(1,:) W(2,:) W(3,:)]';
end

== matlab function Full_Car_Model/SCOPES - 4 MOTORS/MATLAB Function ==
  data: x_b input; y output; end_distance parameter
function y = fcn(x_b, end_distance)
if x_b > end_distance
y = 1;
else
y = 0;
end

== matlab function Full_Car_Model/CONTROLLER REAR RIGHT/Subsystem1/MATLAB Function1 ==
  data: QN1 input; WNmat_NMPC output; QN2 input
function WNmat_NMPC = fcn(QN1, QN2) 
     WN                  = diag([QN1 QN2]);
     WNmat_NMPC  = [WN(1,:) WN(2,:)]'; 
    % WN                  = diag([QN1]);
    % WNmat_NMPC  = [WN(1,:) WN(2,:)]'; 
end

== matlab function Full_Car_Model/CONTROLLER FRONT RIGHT/Subsystem2/MATLAB Function ==
  data: Q1 input; Wmat_NMPC output; Q2 input; R1 input; R2 input
function Wmat_NMPC = fcn(Q1, Q2, R1, R2) 
    W = diag([Q1 Q2 R1 R2]);
    Wmat_NMPC   = [W(1,:) W(2,:) W(3,:) W(4,:)]';
end

== matlab function Full_Car_Model/CONTROLLER FRONT RIGHT/Subsystem2/MATLAB Function1 ==
  data: QN1 input; WNmat_NMPC output; QN2 input
function WNmat_NMPC = fcn(QN1, QN2) 
    WN                  = diag([QN1 QN2]);
    WNmat_NMPC  = [WN(1,:) WN(2,:)]'; 
    % WN                  = diag([QN1]);
    % WNmat_NMPC  = [WN(1,:) WN(2,:)]'; 
end

== matlab function Full_Car_Model/CONTROLLER REAR LEFT/Subsystem2/MATLAB Function ==
  data: Q1 input; Wmat_NMPC output; Q2 input; R1 input; R2 input
function Wmat_NMPC = fcn(Q1, Q2, R1, R2) 
    W = diag([Q1 Q2 R1 R2]);
    Wmat_NMPC   = [W(1,:) W(2,:) W(3,:) W(4,:)]';
end

== matlab function Full_Car_Model/CONTROLLER REAR LEFT/Subsystem2/MATLAB Function1 ==
  data: QN1 input; WNmat_NMPC output; QN2 input
function WNmat_NMPC = fcn(QN1, QN2) 
    WN                  = diag([QN1 QN2]);
    WNmat_NMPC  = [WN(1,:) WN(2,:)]'; 
    % WN                  = diag([QN1]);
    % WNmat_NMPC  = [WN(1,:) WN(2,:)]'; 
end

== matlab function Full_Car_Model/CONTROLLER REAR RIGHT/Subsystem2/MATLAB Function ==
  data: Q1 input; Wmat_NMPC output; Q2 input; R1 input; R2 input
function Wmat_NMPC = fcn(Q1, Q2, R1, R2) 
     W = diag([Q1 Q2 R1 R2]);
     Wmat_NMPC   = [W(1,:) W(2,:) W(3,:) W(4,:)]';
end

== matlab function Full_Car_Model/CONTROLLER FRONT RIGHT/MATLAB Function ==
  data: z_b_dot input; z_b_dot_F output; z_b input; z_u_dot_F_R input; z_u_F_R input; x_b_dot input; x_b input; x_u_dot_F_R input; x_u_F_R input; theta_w_dot input; theta_w input; theta_s_dot input; theta_s input; z_b_F output; z_u_dot_F_R output; z_u_F_R output; x_b_dot_F output; x_b_F output; x_u_dot_F_R output; x_u_F_R output; theta_w_dot output; theta_w output; theta_s_dot output; theta_s output; torque input; torque output; pitch_dot input; pitch input; a input
function [z_b_dot_F, z_b_F, z_u_dot_F_R, z_u_F_R,...
          x_b_dot_F, x_b_F, x_u_dot_F_R, x_u_F_R,...
          theta_w_dot, theta_w, theta_s_dot, theta_s, torque]...
          = fcn(z_b_dot, z_b, z_u_dot_F_R, z_u_F_R,...
                x_b_dot, x_b, x_u_dot_F_R, x_u_F_R,...
                theta_w_dot, theta_w, theta_s_dot, theta_s, torque,...
                pitch_dot, pitch,a)

z_b_dot_F   = z_b_dot + pitch_dot*a;
z_b_F       = z_b + a*tan(pitch);
x_b_dot_F   = x_b_dot;
x_b_F       = x_b + a;

end

== matlab function Full_Car_Model/CONTROLLER REAR RIGHT/Subsystem2/MATLAB Function1 ==
  data: QN1 input; WNmat_NMPC output; QN2 input
function WNmat_NMPC = fcn(QN1, QN2) 
    WN                  = diag([QN1 QN2]);
    WNmat_NMPC  = [WN(1,:) WN(2,:)]'; 
    % WN                  = diag([QN1]);
    % WNmat_NMPC  = [WN(1,:) WN(2,:)]'; 
end

== matlab function Full_Car_Model/CONTROLLER FRONT LEFT/Subsystem1/MATLAB Function ==
  data: Q1 input; Wmat_NMPC output; Q2 input; R1 input; R2 input
function Wmat_NMPC = fcn(Q1, Q2, R1, R2) 
     W = diag([Q1 Q2 R1 R2]);
     Wmat_NMPC   = [W(1,:) W(2,:) W(3,:) W(4,:)]';
    % W = diag([Q1 R1 R2]);
    % Wmat_NMPC   = [W(1,:) W(2,:) W(3,:)]';
end

== matlab function Full_Car_Model/CONTROLLER FRONT LEFT/Subsystem1/MATLAB Function1 ==
  data: QN1 input; WNmat_NMPC output; QN2 input
function WNmat_NMPC = fcn(QN1, QN2) 
     WN                  = diag([QN1 QN2]);
     WNmat_NMPC  = [WN(1,:) WN(2,:)]'; 
    % WN                  = diag([QN1]);
    % WNmat_NMPC  = [WN(1,:) WN(2,:)]'; 
end

== matlab function Full_Car_Model/CONTROLLER FRONT LEFT/Subsystem2/MATLAB Function ==
  data: Q1 input; Wmat_NMPC output; Q2 input; R1 input; R2 input
function Wmat_NMPC = fcn(Q1, Q2, R1, R2) 
    W = diag([Q1 Q2 R1 R2]);
    Wmat_NMPC   = [W(1,:) W(2,:) W(3,:) W(4,:)]';
end

== matlab function Full_Car_Model/CONTROLLER FRONT LEFT/Subsystem2/MATLAB Function1 ==
  data: QN1 input; WNmat_NMPC output; QN2 input
function WNmat_NMPC = fcn(QN1, QN2) 
    WN                  = diag([QN1 QN2]);
    WNmat_NMPC  = [WN(1,:) WN(2,:)]'; 
    % WN                  = diag([QN1]);
    % WNmat_NMPC  = [WN(1,:) WN(2,:)]'; 
end

== matlab function Full_Car_Model/CONTROLLER FRONT RIGHT/Rule based/Subsystem/MATLAB Function ==
  data: OnlineData input; w output; M parameter; mu_act output
function [w, mu_act]=fcn(OnlineData, M)

w=zeros(M+1,1);
mu_act=zeros(M+1,1);

for i = 1:M+1       % M = Time preview steps
    w(i) = OnlineData(8*i-7);
    mu_act(i) = OnlineData(8*i-1);
end

== matlab function Full_Car_Model/NMPC Internal model FL/Time-based Road Preview/MATLAB Function1 ==
  data: z_road input; Z_ef output; Z_er output; data parameter
function [Z_ef, Z_er] = fcn(z_road, data)

n_ellipse_width = length(-data.ac:0.01:data.ac);
x_ef = -data.ac:data.ac_step:data.ac;
x_er = x_ef;

Z_ef = max(z_road(end-n_ellipse_width+1:end)' + abs(data.bc*(1-(abs(x_ef)/data.ac).^data.c).^(1/data.c)));
Z_er = max(z_road(1:n_ellipse_width)' + abs(data.bc*(1-(abs(x_er)/data.ac).^data.c).^(1/data.c)));

== matlab function Full_Car_Model/NMPC Internal model FL/Time-based Road Preview/MATLAB Function4 ==
  data: Z_ef input; w output; Z_er input; beta_y output; data parameter
function [w, beta_y] = fcn(Z_ef, Z_er,data)

w = (Z_ef + Z_er)/2 - data.bc;
beta_y = atan((Z_ef - Z_er)/data.ls);

== matlab function Full_Car_Model/CONTROLLER FRONT RIGHT/Weight matrixes/MATLAB Function ==
  data: Q1 input; Wmat_NMPC output; Q2 input; QN1 input; QN2 input; R1 input; R2 input; WNmat_NMPC output
function [Wmat_NMPC,WNmat_NMPC] = fcn(Q1, Q2, QN1, QN2, R1, R2) 
W                   = diag([Q1 Q2 R1 R2]);
WN                  = diag([QN1 QN2]);
Wmat_NMPC   = [W(1,:) W(2,:) W(3,:) W(4,:)]';
WNmat_NMPC  = [WN(1,:) WN(2,:)]';
end

== matlab function Full_Car_Model/CONTROLLER REAR LEFT/Rule based/Subsystem/MATLAB Function ==
  data: OnlineData input; w output; M parameter; mu_act output
function [w, mu_act]=fcn(OnlineData, M)

w=zeros(M+1,1);
mu_act=zeros(M+1,1);

for i = 1:M+1       % M = Time preview steps
    w(i) = OnlineData(8*i-7);
    mu_act(i) = OnlineData(8*i-1);
end

== matlab function Full_Car_Model/CONTROLLER REAR RIGHT/Rule based/Subsystem/MATLAB Function ==
  data: OnlineData input; w output; M parameter; mu_act output
function [w, mu_act]=fcn(OnlineData, M)

w=zeros(M+1,1);
mu_act=zeros(M+1,1);

for i = 1:M+1       % M = Time preview steps
    w(i) = OnlineData(8*i-7);
    mu_act(i) = OnlineData(8*i-1);
end

== matlab function Full_Car_Model/CONTROLLER FRONT RIGHT/Rule based/MATLAB Function ==
  data: w_prev input; W output; w1_h0 parameter; w1_k parameter; w1_max parameter; w1_min parameter; mu input; w1_sat parameter
function W = fcn(w_prev,w1_h0, w1_k, w1_max, w1_min, mu, w1_sat)
h=0;

w_var=zeros(1,length(w_prev)-1);

x1 = linspace(0, 1, length(w_prev)-1);
exp_growth = exp(1 * x1) - 1;   
perc = exp_growth / sum(exp_growth);

for i=1:length(w_prev)-1
    w_var(i)=abs(w_prev(i+1)-w_prev(i)); 
    h=h+w_var(i)*perc(i);
end
W=w1_min+(w1_max-w1_min)/(1+exp(-w1_k*(abs(h)-w1_h0)));

% Saturation between - w1_min and W. The larger is w1_sat, the more is saturated
W = (W - w1_min)*mu^w1_sat + w1_min;

== matlab function Full_Car_Model/CONTROLLER FRONT RIGHT/Rule based/MATLAB Function2 ==
  data: dT_req input; W output; w2_min parameter; w2_max parameter; w2_k parameter; w2_h0 parameter; mu input; w2_inc parameter
function W = fcn(dT_req, w2_min, w2_max, w2_k, w2_h0, mu, w2_inc)
h=0;

x1 = linspace(0, 1, length(dT_req));
exp_decay = exp(5 * x1) - 1;  
perc = exp_decay / sum(exp_decay);

for i=1:length(dT_req)
    h=h+dT_req(i)*perc(i);
end
W=w2_min+(w2_max-w2_min)/(1+exp(-w2_k*(abs(h)-w2_h0)));

% The larger is w2_inc, the more W is incremented
W = (W - w2_min)/(mu^w2_inc) + w2_min;

== matlab function Full_Car_Model/CONTROLLER FRONT RIGHT/Rule based/MATLAB Function3 ==
  data: flag input; mu_prev input; W output; M parameter; r1_min parameter; r1_max parameter; r1_k parameter; r1_h0 parameter
function W = fcn(flag, mu_prev,M, r1_min, r1_max, r1_k, r1_h0)
h=0; 

x2 = linspace(0, 1, M+1);    
exp_growth = exp(1 * x2) - 1;  

perc = exp_growth; 
perc = perc / sum(perc);

for i=1:M+1
    h=h+mu_prev(i)*perc(i);
end

W=r1_min+(r1_max-r1_min)/(1+exp(r1_k*(abs(h)-r1_h0)));

if not(flag)
    W = r1_min;
end

== matlab function Full_Car_Model/CONTROLLER REAR RIGHT/Rule based/MATLAB Function ==
  data: w_prev input; W output; w1_h0 parameter; w1_k parameter; w1_max parameter; w1_min parameter; mu input; w1_sat parameter
function W = fcn(w_prev,w1_h0, w1_k, w1_max, w1_min, mu, w1_sat)
h=0;

w_var=zeros(1,length(w_prev)-1);

x1 = linspace(0, 1, length(w_prev)-1);
exp_growth = exp(1 * x1) - 1;   
perc = exp_growth / sum(exp_growth);

for i=1:length(w_prev)-1
    w_var(i)=abs(w_prev(i+1)-w_prev(i)); 
    h=h+w_var(i)*perc(i);
end
W=w1_min+(w1_max-w1_min)/(1+exp(-w1_k*(abs(h)-w1_h0)));

% Saturation between - w1_min and W. The larger is w1_sat, the more is saturated
W = (W - w1_min)*mu^w1_sat + w1_min;

== matlab function Full_Car_Model/CONTROLLER REAR RIGHT/Rule based/MATLAB Function2 ==
  data: dT_req input; W output; w2_min parameter; w2_max parameter; w2_k parameter; w2_h0 parameter; mu input; w2_inc parameter
function W = fcn(dT_req, w2_min, w2_max, w2_k, w2_h0, mu, w2_inc)
h=0;

x1 = linspace(0, 1, length(dT_req));
exp_decay = exp(5 * x1) - 1;  
perc = exp_decay / sum(exp_decay);

for i=1:length(dT_req)
    h=h+dT_req(i)*perc(i);
end
W=w2_min+(w2_max-w2_min)/(1+exp(-w2_k*(abs(h)-w2_h0)));

% The larger is w2_inc, the more W is incremented
W = (W - w2_min)/(mu^w2_inc) + w2_min;

== matlab function Full_Car_Model/CONTROLLER REAR RIGHT/Rule based/MATLAB Function3 ==
  data: flag input; mu_prev input; W output; M parameter; r1_min parameter; r1_max parameter; r1_k parameter; r1_h0 parameter
function W = fcn(flag, mu_prev,M, r1_min, r1_max, r1_k, r1_h0)
h=0; 

x2 = linspace(0, 1, M+1);    
exp_growth = exp(1 * x2) - 1;  

perc = exp_growth; 
perc = perc / sum(perc);

for i=1:M+1
    h=h+mu_prev(i)*perc(i);
end

W=r1_min+(r1_max-r1_min)/(1+exp(r1_k*(abs(h)-r1_h0)));

if not(flag)
    W = r1_min;
end

== matlab function Full_Car_Model/CONTROLLER FRONT LEFT/Rule based/MATLAB Function ==
  data: w_prev input; W output; w1_h0 parameter; w1_k parameter; w1_max parameter; w1_min parameter; mu input; w1_sat parameter
function W = fcn(w_prev,w1_h0, w1_k, w1_max, w1_min, mu, w1_sat)
h=0;

w_var=zeros(1,length(w_prev)-1);

x1 = linspace(0, 1, length(w_prev)-1);
exp_growth = exp(1 * x1) - 1;   
perc = exp_growth / sum(exp_growth);

for i=1:length(w_prev)-1
    w_var(i)=abs(w_prev(i+1)-w_prev(i)); 
    h=h+w_var(i)*perc(i);
end
W=w1_min+(w1_max-w1_min)/(1+exp(-w1_k*(abs(h)-w1_h0)));

% Saturation between - w1_min and W. The larger is w1_sat, the more is saturated
W = (W - w1_min)*mu^w1_sat + w1_min;

== matlab function Full_Car_Model/CONTROLLER FRONT LEFT/Subsystem1/MATLAB Function2 ==
  data: Q1 input; mu input; Q1_out output; LowLim_Q1 parameter; Q1_sat parameter
function Q1_out = fcn(Q1, mu, LowLim_Q1, Q1_sat)

% Saturation between - w1_min and W. The larger is w1_sat, the more is saturated
Q1_out = (Q1 - LowLim_Q1)*mu^Q1_sat + LowLim_Q1;

== matlab function Full_Car_Model/CONTROLLER FRONT RIGHT/Subsystem1/MATLAB Function2 ==
  data: Q1 input; mu input; Q1_out output; LowLim_Q1 parameter; Q1_sat parameter
function Q1_out = fcn(Q1, mu, LowLim_Q1, Q1_sat)

% Saturation between - w1_min and W. The larger is w1_sat, the more is saturated
Q1_out = (Q1 - LowLim_Q1)*mu^Q1_sat + LowLim_Q1;

== matlab function Full_Car_Model/CONTROLLER REAR LEFT/Weight matrixes/MATLAB Function ==
  data: Q1 input; Wmat_NMPC output; Q2 input; QN1 input; QN2 input; R1 input; R2 input; WNmat_NMPC output
function [Wmat_NMPC,WNmat_NMPC] = fcn(Q1, Q2, QN1, QN2, R1, R2) 
W                   = diag([Q1 Q2 R1 R2]);
WN                  = diag([QN1 QN2]);
Wmat_NMPC   = [W(1,:) W(2,:) W(3,:) W(4,:)]';
WNmat_NMPC  = [WN(1,:) WN(2,:)]';
end

== matlab function Full_Car_Model/CONTROLLER REAR RIGHT/Weight matrixes/MATLAB Function ==
  data: Q1 input; Wmat_NMPC output; Q2 input; QN1 input; QN2 input; R1 input; R2 input; WNmat_NMPC output
function [Wmat_NMPC,WNmat_NMPC] = fcn(Q1, Q2, QN1, QN2, R1, R2) 
W                   = diag([Q1 Q2 R1 R2]);
WN                  = diag([QN1 QN2]);
Wmat_NMPC   = [W(1,:) W(2,:) W(3,:) W(4,:)]';
WNmat_NMPC  = [WN(1,:) WN(2,:)]';
end

== matlab function Full_Car_Model/CONTROLLER REAR LEFT/Subsystem1/MATLAB Function2 ==
  data: Q1 input; mu input; Q1_out output; LowLim_Q1 parameter; Q1_sat parameter
function Q1_out = fcn(Q1, mu, LowLim_Q1, Q1_sat)

% Saturation between - w1_min and W. The larger is w1_sat, the more is saturated
Q1_out = (Q1 - LowLim_Q1)*mu^Q1_sat + LowLim_Q1;

== matlab function Full_Car_Model/CONTROLLER FRONT RIGHT/ROAD PREVIEW/NO_ROAD_PREVIEW ==
  data: w input; OnlineData output; Tm_req input; Tm_req_F2 input; Tm_req_R_L input; Tm_req_R_R input; N parameter; mu_act input; sigma_ref input
function OnlineData=OnlineDataArray(w, Tm_req, Tm_req_F2, Tm_req_R_L, Tm_req_R_R, N, mu_act, sigma_ref)

OnlineData = repmat([w; 0; Tm_req; Tm_req_F2; Tm_req_R_L; Tm_req_R_R; mu_act; sigma_ref],N+1,1);
end

== matlab function Full_Car_Model/CONTROLLER FRONT RIGHT/ROAD PREVIEW/ROAD PREVIEW ==
  data: w input; OnlineData output; beta_y input; Tm_req input; Tm_req_F2 input; Tm_req_R_L input; Tm_req_R_R input; N parameter; M parameter; mu_act input; sigma_ref input
function OnlineData=OnlineDataArray(w, beta_y, Tm_req, Tm_req_F2, Tm_req_R_L, Tm_req_R_R, N, M, mu_act, sigma_ref)

OnlineData = repmat([0; 0; Tm_req; Tm_req_F2; Tm_req_R_L; Tm_req_R_R; 0; 0],N+1,1);

for i = 1:M+1       % M = Time preview steps
    OnlineData(8*i-7) = w(i);
    OnlineData(8*i-6) = beta_y(i);
    OnlineData(8*i-1) = mu_act(i);
    OnlineData(8*i) = sigma_ref(i);
end

for i = M+2:N+1     % N = Time horizon steps
    OnlineData(8*i-7) = w(end);
    OnlineData(8*i-6) = beta_y(end);
    OnlineData(8*i-1) = mu_act(end);
    OnlineData(8*i) = sigma_ref(end);

end

== matlab function Full_Car_Model/CONTROLLER FRONT RIGHT/ROAD PREVIEW/Time-based Road Preview/MATLAB Function2 ==
  data: z_road input; Z_ef output; Z_er output; data parameter; M parameter
function [Z_ef, Z_er] = fcn(z_road, data, M)

n_ellipse_width = length(-data.ac:0.01:data.ac);
x_ef = -data.ac:data.ac_step:data.ac;
x_er = x_ef;

Z_ef = zeros(M+1,1);
Z_er = zeros(M+1,1);
for i = 1:M+1
    Z_ef(i) = max(z_road(i,end-n_ellipse_width+1:end) + abs(data.bc*(1-(abs(x_ef)/data.ac).^data.c).^(1/data.c)));
    Z_er(i) = max(z_road(i,1:n_ellipse_width) + abs(data.bc*(1-(abs(x_er)/data.ac).^data.c).^(1/data.c)));
end

== matlab function Full_Car_Model/CONTROLLER FRONT RIGHT/ROAD PREVIEW/Time-based Road Preview/MATLAB Function3 ==
  data: Z_ef input; w output; Z_er input; beta_y output; data parameter; M parameter
function [w, beta_y] = fcn(Z_ef, Z_er,data, M)

w      = zeros(M+1,1);
beta_y = zeros(M+1,1);

for i = 1:M+1
    w(i) = (Z_ef(i) + Z_er(i))/2 - data.bc;
    beta_y(i) = atan((Z_ef(i) - Z_er(i))/data.ls);
end

== matlab function Full_Car_Model/CONTROLLER FRONT RIGHT/ROAD PREVIEW/Time-based Road Preview/MATLAB Function6 ==
  data: X_i input; X_road output; M parameter; data parameter
function X_road = fcn(X_i, M, data)

n = length(0:0.01:data.ac*2+data.ls);

X_road = zeros(M+1, n+1);

for i=1:M+1
    for j=1:1:n+1
        X_road(i,j) = X_i(i) - data.ls/2 - data.ac + data.ac_step*(j-1);
    end
end

== matlab function Full_Car_Model/CONTROLLER FRONT LEFT/Reference Generation ==
  data: a_b_ref input; References output; N parameter; data parameter
function References    = fcn(a_b_ref, N, data)

 href=[a_b_ref 0 0 0];                      
 References_horizon = [repmat(href,N,1)].';
 hN = [a_b_ref 0];
 References_end = hN.';

References=[References_horizon(:); References_end(:)];
end

== matlab function Full_Car_Model/CONTROLLER FRONT RIGHT/ROAD PREVIEW/Time-based Road Preview/X(i)1 ==
  data: X_i output; X_u_current input; x_u_dot_current input; Ts parameter; M parameter
function X_i= fcn(X_u_current, x_u_dot_current, Ts, M)

X_i = zeros(M+1,1);

for i=1:M+1
    X_i(i) = X_u_current + x_u_dot_current * Ts(i);
end

== matlab function Full_Car_Model/CONTROLLER FRONT RIGHT/Reference Generation ==
  data: a_b_ref input; References output; N parameter; data parameter
function References    = fcn(a_b_ref, N, data)

 href=[a_b_ref 0 0 0];                      
 References_horizon = [repmat(href,N,1)].';
 hN = [a_b_ref 0];
 References_end = hN.';

References=[References_horizon(:); References_end(:)];
end

== matlab function Full_Car_Model/CONTROLLER REAR RIGHT/Subsystem1/MATLAB Function2 ==
  data: Q1 input; mu input; Q1_out output; LowLim_Q1 parameter; Q1_sat parameter
function Q1_out = fcn(Q1, mu, LowLim_Q1, Q1_sat)

% Saturation between - w1_min and W. The larger is w1_sat, the more is saturated
Q1_out = (Q1 - LowLim_Q1)*mu^Q1_sat + LowLim_Q1;
